simulink model "FAFA_Simulation"  (R2024b)
settings: Solver=FixedStepAuto  StartTime=0.0  StopTime=250  FixedStep=0.1  RelTol=1e-3
model workspace (MAT data in the model file):
  E = 0
  N = 0
  U = 70
  a_lat = [-2.8994 -3.7694 4.8979 0.9075 0.2017 1.1605 -2.4536 1.8506 -1.4522 0.9879 -4.2099 6.4665 ... (16 elements, 4x4)]
  a_lon = [-0.1636 0.8185 -0.1448 0.6823 -0.7164 -0.2899 -2.0395 -2.5415 0.3908 2.1971 -0.2446 -6.117 ... (16 elements, 4x4)]
  b_lat = [-2.6641  1.8404; -6.8743  1.3852; 17.3529  -0.0089; -11.8089  -3.3692]
  b_lon = [1.3105; 2.2437; -0.9608; -9.211]
  c_lat = [-0.6923 -1.1619 0.5476 -0.4273 0.0805 0.5751 0.4203 0.7792 -0.3221 1.1098 0.2079 0.2479 ... (16 elements, 4x4)]
  c_lon = [-5.1576 -0.0952 0.5331 3.6707 -28.9963 -0.3715 -3.4973 -0.1414 19.7487 -0.0997 -0.5832 -0.2256 ... (16 elements, 4x4)]
  d_lat = [0  0; 0  0; 0  0; 0  0]
  d_lon = [0; 0; 0; 0]
  psi0 = 0
  wind_E0 = 0
  wind_N0 = 0
  wind_heading = 100
  wind_noise = 0
  wind_turbulance_value0 = 1
  wind_value0 = 0
  x0_lat = [0; 0; 0; 0]
  x0_lon = [0; 0; 0; 0]
values from neighbouring files (symbols this model uses):
  velocity = zeros(num_waypoints, 3)    [training_engine.m]
  waypoints = all_waypoints    [training_engine.m]
undefined symbols (not defined in the file or in its folder): dspblkCoreblockFVToolHelper, F, gcbh, Light, MIL
libraries: simulink x8, slpidlib x5, aerolibwind2 x3, sharedtransform x2, rllib x1, uavutilslib x1
(part 3 of 3)

== matlab function FAFA_Simulation/OBSERVATION/Straight Line V4 ==
  data: waypoints_window input; velocity_window input; valid_flag input; loiter_flag input; uav_e input; global_path output size=[inf 3]; uav_n input; uav_u input; guidance_mode output; uav_phi input; uav_theta input; uav_psi input; debug_cte output; debug_curvature output
function [global_path, guidance_mode, debug_cte, debug_curvature] = guidance_function_hybrid_Straight_Line(waypoints_window, velocity_window, valid_flag, loiter_flag, uav_e, uav_n, uav_u, uav_phi, uav_theta, uav_psi)
% guidance_mode: 0=無效, 1=純B-spline, 2=SPSO+B-spline, 3=Loiter模式
%#codegen

%  Loiter 模式開關
ENABLE_LOITER = false;

persistent last_point_initialized last_point stored_global_path stored_path_length ...
           loiter_mode initialized theta_current center loiter_arc transition ...
           a1_mode_active

if isempty(last_point_initialized)
    last_point_initialized = false;
    last_point            = zeros(1,3);
    stored_global_path    = zeros(100000,3);
    stored_path_length    = 1;
    loiter_mode           = false;
    initialized = false;
    theta_current = 0;
    center = [0 0];
    loiter_arc = zeros(3,3);
    transition = false;
    a1_mode_active = false;
end

% 確保輸出在所有路徑都有明確的標量值
guidance_mode = 0;
debug_cte = 0;
debug_curvature = 0;

R = 100;
dtheta_deg = 1;
uav_position = [uav_e, uav_n, uav_u];

%% ==== Loiter 模式 ====
% 只有當 ENABLE_LOITER = true 時才會進入 Loiter 邏輯
if ENABLE_LOITER && loiter_flag && ~initialized
    if stored_path_length >= 2
        pos_prev = stored_global_path(stored_path_length-1, 1:2);
        pos_curr = stored_global_path(stored_path_length, 1:2);
        heading_vec = pos_curr - pos_prev;
        yaw = atan2(heading_vec(2), heading_vec(1));
    else
        yaw = 0;
    end

    dists = vecnorm(waypoints_window(:,1:2) - uav_position(1:2), 2, 2);
    [~, idx_nearest] = min(dists);
    P0 = waypoints_window(idx_nearest, 1:2);
    center = P0 + [cos(yaw), sin(yaw)] * R * 1.5;
    theta_current = atan2(uav_position(2) - center(2), ...
                           uav_position(1) - center(1));
    loiter_mode = true;
    initialized = true;
end

if ENABLE_LOITER && loiter_mode
    guidance_mode = 3;
    a1_mode_active = false;

    if loiter_flag
        dtheta = deg2rad(dtheta_deg);
        spacing = 1.0;
        arc_length = R * dtheta;
        num_points = max(3, ceil(arc_length / spacing));
        theta_list = theta_current - linspace(0, dtheta, num_points);
        x_list = center(1) + R * cos(theta_list);
        y_list = center(2) + R * sin(theta_list);
        z_list = repmat(uav_u, size(x_list));

        loiter_arc_raw = [x_list', y_list', z_list'];
        arc_diff = diff(loiter_arc_raw);
        arc_seg_length = sqrt(sum(arc_diff.^2, 2));
        cum_length = [0; cumsum(arc_seg_length)];
        total_length = cum_length(end);

        num_interp = max(2, ceil(total_length));
        query_dist = linspace(0, total_length, num_interp)';
        interp_x = interp1(cum_length, loiter_arc_raw(:,1), query_dist, 'linear');
        interp_y = interp1(cum_length, loiter_arc_raw(:,2), query_dist, 'linear');
        interp_z = interp1(cum_length, loiter_arc_raw(:,3), query_dist, 'linear');
        loiter_arc = [interp_x, interp_y, interp_z];
        theta_current = theta_list(end);

        if ~transition
            loiter_entry = loiter_arc(1,:);
            loiter_tangent = loiter_arc(2,1:2) - loiter_arc(1,1:2);
            loiter_tangent = loiter_tangent / (norm(loiter_tangent) + 1e-6);

            dists = vecnorm(waypoints_window(:,1:2) - uav_position(1:2), 2, 2);
            [~, idx_nearest] = min(dists);
            P0 = waypoints_window(idx_nearest, :);

            connect_tangent = loiter_entry(1:2) - P0(1:2);
            connect_tangent = connect_tangent / (norm(connect_tangent) + 1e-6);
            dist = norm(loiter_entry(1:2) - P0(1:2));

            P1 = P0(1:2) + 0.3 * dist * connect_tangent;
            P2 = loiter_entry(1:2) - 0.3 * dist * loiter_tangent;
            P3 = loiter_entry(1:2);

            t = linspace(0,1,ceil(dist));
            bezier_x = (1-t).^3 * P0(1) + 3*(1-t).^2 .* t * P1(1) + 3*(1-t).*t.^2 * P2(1) + t.^3 * P3(1);
            bezier_y = (1-t).^3 * P0(2) + 3*(1-t).^2 .* t * P1(2) + 3*(1-t).*t.^2 * P2(2) + t.^3 * P3(2);
            bezier_z = linspace(P0(3), loiter_entry(3), numel(t));
            transition_path = [bezier_x', bezier_y', bezier_z'];

            combined_path = [transition_path; loiter_arc(2:end,:)];
            global_path = combined_path;
            transition = true;
        else
            global_path = loiter_arc;
        end
        return;
    else
        % 退出 Loiter 的邏輯
        arc_exit_pt = loiter_arc(end, :);
        arc_tangent = loiter_arc(end,1:2) - loiter_arc(end-1,1:2);
        arc_tangent = arc_tangent / (norm(arc_tangent) + 1e-6);
        R_min = 55;
        dists = vecnorm(waypoints_window(:,1:2) - arc_exit_pt(1:2), 2, 2);
        [~, idx_nearest] = min(dists);
        lookahead_distance = 100;
        accum_dist = 0;
        idx_target = idx_nearest;

        while accum_dist < lookahead_distance && idx_target < size(waypoints_window,1)
            delta = norm(waypoints_window(idx_target+1,1:2) - waypoints_window(idx_target,1:2));
            accum_dist = accum_dist + delta;
            idx_target = idx_target + 1;
        end

        p_target = waypoints_window(idx_target, :);

        if idx_target < size(waypoints_window,1)
            next_vec = waypoints_window(idx_target+1,1:2) - waypoints_window(idx_target,1:2);
        else
            next_vec = waypoints_window(idx_target,1:2) - waypoints_window(idx_target-1,1:2);
        end

        target_tangent = next_vec / (norm(next_vec) + 1e-6);
        P0 = arc_exit_pt;
        P3 = p_target;
        total_dist = norm(P3(1:2) - P0(1:2));
        theta = acos(dot(arc_tangent, target_tangent));
        d_min = R_min * tan(theta/2);
        d = max(d_min, R_min);
        success = false;
        B = repmat(P0, ceil(total_dist), 1);

        while ~success && d <= total_dist
            P1 = P0 + [arc_tangent, 0] * 0.3 * d;
            P2 = P3 - [target_tangent, 0] * 0.1 * d;
            t = linspace(0,1,ceil(total_dist));
            B = (1 - t').^3 * P0 + 3*(1 - t').^2 .* t' * P1 + 3*(1 - t') .* t'.^2 * P2 + t'.^3 * P3;
            d1 = diff(B, 1, 1);
            d2 = diff(d1, 1, 1);
            cross_z = d1(1:end-1,1) .* d2(:,2) - d1(1:end-1,2) .* d2(:,1);
            curvature = abs(cross_z) ./ (vecnorm(d1(1:end-1,:),2,2).^3 + 1e-6);

            if all(1./(curvature + 1e-6) >= R_min)
                success = true;
            else
                d = d + 5;
            end
        end

        segment = B;
        stored_global_path(1:size(segment,1), :) = segment;
        stored_path_length = size(segment,1);
        loiter_mode = false;
        initialized = false;
        transition = false;
        global_path = segment;

        % 固定維度賦值
        if size(segment,1) >= 1
            last_point(1,1) = segment(end, 1);
            last_point(1,2) = segment(end, 2);
            last_point(1,3) = segment(end, 3);
        end
        return;
    end
end

%% ========== v8 混合規劃器 ==========
if valid_flag && ~loiter_mode

    N_WAYPOINTS = size(waypoints_window, 1);

    % 起點處理
    if ~last_point_initialized
        P_start_spline = [uav_e, uav_n, uav_u];
        last_point_initialized = true;
    else
        P_start_spline = last_point;
    end

    P_end = waypoints_window(end, :);

    % ====== 計算 UAV 到滑窗的真正 CTE（垂直投影距離） ======
    uav_cte = inf;
    if N_WAYPOINTS >= 2
        for i = 1:N_WAYPOINTS-1
            seg_s = waypoints_window(i, 1:2);
            seg_e = waypoints_window(i+1, 1:2);
            seg_v = seg_e - seg_s;
            seg_l = norm(seg_v);
            if seg_l < 1e-6, continue; end
            to_uav = uav_position(1:2) - seg_s;
            proj = max(0, min(1, dot(to_uav, seg_v) / (seg_l^2)));
            d = norm(uav_position(1:2) - (seg_s + proj * seg_v));
            if d < uav_cte, uav_cte = d; end
        end
    end

    % 點到點距離（用於 A-2 和 SPSO 判斷）
    dists_to_window = vecnorm(waypoints_window(:,1:2) - uav_position(1:2), 2, 2);
    [min_dist_to_window, ~] = min(dists_to_window);
    dist_start_to_window = norm(P_start_spline(1:2) - waypoints_window(1,1:2));

    % ====== 計算滑窗最大曲率 (Menger curvature) ======
    max_curvature = 0;
    if N_WAYPOINTS >= 3
        for i = 2:N_WAYPOINTS-1
            AB = waypoints_window(i,1:2) - waypoints_window(i-1,1:2);
            BC = waypoints_window(i+1,1:2) - waypoints_window(i,1:2);
            AC = waypoints_window(i+1,1:2) - waypoints_window(i-1,1:2);
            cross_z = abs(AB(1)*BC(2) - AB(2)*BC(1));
            denom = norm(AB) * norm(BC) * norm(AC);

            if denom > 1e-10
                kappa = 2 * cross_z / denom;
                if kappa > max_curvature
                    max_curvature = kappa;
                end
            end
        end
    end

    % ====== 計算滑窗平均朝向，並與 UAV 航向比較 ======
    % uav_psi 使用弧度；此處以滑窗各線段向量加總作為平均朝向
    window_avg_vec = [0, 0];
    heading_error = pi;

    if N_WAYPOINTS >= 2
        for i = 1:N_WAYPOINTS-1
            seg_vec_heading = waypoints_window(i+1, 1:2) - waypoints_window(i, 1:2);
            if norm(seg_vec_heading) > 1e-6
                window_avg_vec = window_avg_vec + seg_vec_heading;
            end
        end

        if norm(window_avg_vec) > 1e-6
            window_avg_heading = atan2(window_avg_vec(2), window_avg_vec(1));
            heading_error = atan2(sin(window_avg_heading - uav_psi), ...
                                  cos(window_avg_heading - uav_psi));
        end
    end

    CURVATURE_THRESHOLD = 0.005;   % 曲率門檻 (對應半徑 > 200m)

    % A-1 航向遲滯門檻：
    % 尚未進入 A-1 時，需小於 17 deg 才允許進入；
    % 已在 A-1 時，允許到 23 deg 才退出，避免在 20 deg 附近反覆切換。
    HEADING_ALIGNMENT_CENTER = deg2rad(20);
    HEADING_ALIGNMENT_RANGE  = deg2rad(3);
    HEADING_ENTER_THRESHOLD  = HEADING_ALIGNMENT_CENTER - HEADING_ALIGNMENT_RANGE;  % 17 deg
    HEADING_EXIT_THRESHOLD   = HEADING_ALIGNMENT_CENTER + HEADING_ALIGNMENT_RANGE;  % 23 deg

    CTE_THRESHOLD = 35;            % CTE 門檻 (m)，使用垂直投影距離
    DEVIATION_THRESHOLD = 100;

    % ====== Debug 輸出 ======
    debug_cte = uav_cte;
    debug_curvature = max_curvature;

    % ====== A-1 航向遲滯判斷 ======
    if a1_mode_active
        a1_heading_condition = abs(heading_error) <= HEADING_EXIT_THRESHOLD;
    else
        a1_heading_condition = abs(heading_error) <= HEADING_ENTER_THRESHOLD;
    end

    if max_curvature < CURVATURE_THRESHOLD && a1_heading_condition
        % ========== 模式A-1：低曲率 + 航向對齊 → 純 B-spline (從 UAV 位置出發) ==========
        guidance_mode = 1;
        a1_mode_active = true;
        N_CONTROL_POINTS = 6;
        indices = round(linspace(1, N_WAYPOINTS, N_CONTROL_POINTS));
        best_control_points = waypoints_window(indices, :);
        best_control_points(1, :) = uav_position;  % ★ 從自身位置開始

    elseif min_dist_to_window < DEVIATION_THRESHOLD && dist_start_to_window < DEVIATION_THRESHOLD
        % ========== 模式A-2：原始純 B-spline (從 last_point 出發) ==========
        guidance_mode = 1;
        a1_mode_active = false;
        N_CONTROL_POINTS = 6;
        indices = round(linspace(1, N_WAYPOINTS, N_CONTROL_POINTS));
        best_control_points = waypoints_window(indices, :);
        best_control_points(1, :) = P_start_spline;

    else
        % ========== 模式B：SPSO + B-spline ==========
        guidance_mode = 2;
        a1_mode_active = false;

        % SPSO 起點：強制為 UAV 當前位置
        P_start_SPSO = uav_position;

        % ====== 目標行駛方向（由速度滑窗估計，僅 SPSO 使用） ======
        v_tar_2d = [0, 0];
        if ~isempty(velocity_window)
            N_vel = size(velocity_window, 1);
            if N_vel >= 1
                K = min(3, N_vel);
                idx_start = N_vel - K + 1;
                v_seg = velocity_window(idx_start:N_vel, 1:2);
                v_mean = mean(v_seg, 1);
                if norm(v_mean) > 1e-3
                    v_tar_2d = v_mean;
                else
                    v_tar_2d = [0, 0];
                end
            end
        end

        % SPSO參數
        nParticles = 10;
        maxIter = 20;
        w = 0.4;
        c1 = 1.5;
        c2 = 1.5;

        N_CONTROL_POINTS = 5;
        N_OPTIMIZE = 3;

        max_segment_length = 50;
        min_segment_length = 5;
        max_climb_angle_rad = deg2rad(20);
        max_turn_angle_rad  = deg2rad(35);

        b1 = 0.6;
        b2 = 0.2;
        b3 = 0.1;
        b4 = 0.1;

        % 參考採樣
        sample_idx = round(linspace(1, N_WAYPOINTS, N_CONTROL_POINTS));
        control_waypoints = waypoints_window(sample_idx, :);

        % 初始化參考向量
        reference_vectors = control_waypoints - P_start_SPSO;
        rho_ref = vecnorm(reference_vectors, 2, 2);
        theta_ref = asin(reference_vectors(:,3) ./ (rho_ref + 1e-6));
        phi_ref = atan2(reference_vectors(:,2), reference_vectors(:,1));

        dim = N_OPTIMIZE * 3;
        particles = zeros(nParticles, dim);
        velocities = zeros(nParticles, dim);

        for i = 1:nParticles
            for j = 1:N_OPTIMIZE
                ref_idx = j + 1;
                idx = (j-1)*3 + 1;

                if i == 1
                    particles(1, idx)   = rho_ref(ref_idx);
                    particles(1, idx+1) = theta_ref(ref_idx);
                    particles(1, idx+2) = phi_ref(ref_idx);
                else
                    particles(i, idx)   = rho_ref(ref_idx) * (1 + randn() * 0.1);
                    particles(i, idx+1) = theta_ref(ref_idx) + randn() * deg2rad(2);
                    particles(i, idx+2) = phi_ref(ref_idx) + randn() * deg2rad(5);
                end

                particles(i, idx) = max(min_segment_length, min(particles(i, idx), max_segment_length));
                particles(i, idx+1) = max(-max_climb_angle_rad, min(particles(i, idx+1), max_climb_angle_rad));

                if j == 1
                    base_heading = uav_psi;
                else
                    prev_phi_idx = (j-2)*3 + 3;
                    base_heading = particles(i, prev_phi_idx);
                end

                dphi = particles(i, idx+2) - base_heading;
                dphi = mod(dphi + pi, 2*pi) - pi;
                if dphi > max_turn_angle_rad
                    dphi = max_turn_angle_rad;
                elseif dphi < -max_turn_angle_rad
                    dphi = -max_turn_angle_rad;
                end
                particles(i, idx+2) = mod(base_heading + dphi + pi, 2*pi) - pi;
            end
            velocities(i, :) = randn(1, dim) * 0.01;
        end

        % SPSO迭代
        fitness = zeros(nParticles, 1);
        for i = 1:nParticles
            fitness(i) = evaluateFitness_CostStruct(particles(i,:), P_start_SPSO, P_end, ...
                          control_waypoints, N_CONTROL_POINTS, b1, b2, b3, b4, ...
                          uav_psi, v_tar_2d);
        end

        [~, best_idx] = min(fitness);
        personal_best = particles;
        personal_best_fitness = fitness;
        global_best = particles(best_idx, :);
        global_best_fitness = fitness(best_idx);

        for iter = 1:maxIter
            for i = 1:nParticles
                r1 = rand(1, dim);
                r2 = rand(1, dim);
                velocities(i,:) = w * velocities(i,:) + ...
                                  c1 * r1 .* (personal_best(i,:) - particles(i,:)) + ...
                                  c2 * r2 .* (global_best - particles(i,:));
                particles(i,:) = particles(i,:) + velocities(i,:);

                for j = 1:N_OPTIMIZE
                    idx = (j-1)*3 + 1;
                    particles(i, idx) = max(min_segment_length, min(particles(i, idx), max_segment_length));
                    particles(i, idx+1) = max(-max_climb_angle_rad, min(particles(i, idx+1), max_climb_angle_rad));

                    phi_idx = idx + 2;
                    if j == 1
                        base_heading = uav_psi;
                    else
                        prev_phi_idx = (j-2)*3 + 3;
                        base_heading = particles(i, prev_phi_idx);
                    end

                    dphi = particles(i, phi_idx) - base_heading;
                    dphi = mod(dphi + pi, 2*pi) - pi;
                    if dphi > max_turn_angle_rad
                        dphi = max_turn_angle_rad;
                    elseif dphi < -max_turn_angle_rad
                        dphi = -max_turn_angle_rad;
                    end
                    particles(i, phi_idx) = mod(base_heading + dphi + pi, 2*pi) - pi;
                end

                fitness(i) = evaluateFitness_CostStruct(particles(i,:), P_start_SPSO, P_end, ...
                              control_waypoints, N_CONTROL_POINTS, b1, b2, b3, b4, ...
                              uav_psi, v_tar_2d);

                if fitness(i) < personal_best_fitness(i)
                    personal_best(i,:) = particles(i,:);
                    personal_best_fitness(i) = fitness(i);
                end
            end

            [current_best_fitness, best_idx] = min(fitness);
            if current_best_fitness < global_best_fitness
                global_best = particles(best_idx, :);
                global_best_fitness = current_best_fitness;
            end
        end

        % 構建最終控制點
        best_control_points = zeros(N_CONTROL_POINTS, 3);
        best_control_points(1, :) = P_start_SPSO;
        best_control_points(end, :) = P_end;

        for j = 1:N_OPTIMIZE
            idx = (j-1)*3 + 1;
            rho   = global_best(idx);
            theta = global_best(idx+1);
            phi   = global_best(idx+2);
            dx = rho * cos(theta) * cos(phi);
            dy = rho * cos(theta) * sin(phi);
            dz = rho * sin(theta);
            best_control_points(j+1, :) = best_control_points(j, :) + [dx, dy, dz];
        end
    end

    % 生成 B-spline
    N_samples = 100;
    path_smooth = generate_Bspline(best_control_points, N_samples);

    % Resample
    segment_diff = diff(path_smooth);
    segment_length = sqrt(sum(segment_diff.^2, 2));
    cumulative_length = [0; cumsum(segment_length)];
    total_length = cumulative_length(end);

    if total_length < 1e-3
        if stored_path_length > 1
             global_path = stored_global_path(1:stored_path_length,:);
        else
             global_path = path_smooth;
        end
        return;
    end

    desired_spacing = 1;
    num_new_points = max(2, floor(total_length / desired_spacing));
    query_distances = linspace(0, total_length, num_new_points)';

    interp_x = interp1(cumulative_length, path_smooth(:,1), query_distances, 'linear');
    interp_y = interp1(cumulative_length, path_smooth(:,2), query_distances, 'linear');
    interp_z = interp1(cumulative_length, path_smooth(:,3), query_distances, 'linear');

    new_path = [interp_x, interp_y, interp_z];
    stored_global_path(:,:) = 0;

    if isempty(new_path)
        stored_global_path(1:size(best_control_points,1),:) = best_control_points;
        stored_path_length = size(best_control_points,1);
        last_point(1,1) = best_control_points(end, 1);
        last_point(1,2) = best_control_points(end, 2);
        last_point(1,3) = best_control_points(end, 3);
    else
        stored_global_path(1:size(new_path,1),:) = new_path;
        stored_path_length = size(new_path,1);
        last_point(1,1) = new_path(end, 1);
        last_point(1,2) = new_path(end, 2);
        last_point(1,3) = new_path(end, 3);
    end
end

global_path = stored_global_path(1:stored_path_length,:);
end

%% ========== B-spline生成器 ==========
function path_smooth = generate_Bspline(control_points, num_samples)
    N = size(control_points, 1);
    if N < 2
        path_smooth = control_points;
        return;
    end
    segment_lengths = sqrt(sum(diff(control_points).^2, 2));
    t_control = [0; cumsum(segment_lengths)];
    valid_idx = [true; segment_lengths > 1e-6];
    if sum(valid_idx) < 2
        path_smooth = repmat(control_points(1,:), num_samples, 1);
        return;
    end
    t_control_valid = t_control(valid_idx);
    control_points_valid = control_points(valid_idx, :);
    if isempty(t_control_valid) || t_control_valid(end) < 1e-6
        path_smooth = repmat(control_points(1,:), num_samples, 1);
        return;
    end
    t_control_valid = t_control_valid / t_control_valid(end);
    t_query = linspace(0, 1, num_samples)';
    x_smooth = spline(t_control_valid, control_points_valid(:,1), t_query);
    y_smooth = spline(t_control_valid, control_points_valid(:,2), t_query);
    z_smooth = spline(t_control_valid, control_points_valid(:,3), t_query);
    path_smooth = [x_smooth, y_smooth, z_smooth];
end

%% ========== Cost Function（含終端入射角約束） ==========
function cost = evaluateFitness_CostStruct(particle, P_start, P_end, control_waypoints, N_control, ...
                                           b1, b2, b3, b4, ...
                                           uav_psi, v_tar_2d)
    % 1. 重建路徑
    path = zeros(N_control, 3);
    path(1, :) = P_start;
    path(end, :) = P_end;

    N_optimize = (N_control - 2);
    for j = 1:N_optimize
        idx = (j-1)*3 + 1;
        rho   = particle(idx);
        theta = particle(idx+1);
        phi   = particle(idx+2);
        dx = rho * cos(theta) * cos(phi);
        dy = rho * cos(theta) * sin(phi);
        dz = rho * sin(theta);
        path(j+1, :) = path(j, :) + [dx, dy, dz];
    end

    % ========== F1: 路徑長度成本 ==========
    path_diff = diff(path);
    segment_lengths = sqrt(sum(path_diff.^2, 2));
    total_length = sum(segment_lengths);
    straight_dist = norm(P_end - P_start);

    if straight_dist > 1e-6
        F1 = total_length / straight_dist;
        F1 = min(F1, 3.0);
    else
        F1 = 1.0;
    end

    % ========== F2: 路徑跟隨成本 ==========
    F2_raw = 0;
    for i = 1:size(path,1)
        dists = vecnorm(control_waypoints - path(i,:), 2, 2);
        [min_dist, ~] = min(dists);
        F2_raw = F2_raw + min_dist^2;
    end
    F2 = F2_raw / (size(path,1) * 100);
    F2 = min(F2, 10.0);

    % ========== F3: 平滑度成本 ==========
    F3_raw = 0;
    max_turn_angle = deg2rad(35);

    % (A) 第一段 vs UAV 航向
    vec_first = path(2,1:2) - path(1,1:2);
    if norm(vec_first) > 1e-6
        current_psi_vec = [cos(uav_psi), sin(uav_psi)];
        dot_val = dot(vec_first/norm(vec_first), current_psi_vec);
        angle_diff_start = acos(max(-1, min(1, dot_val)));
        if angle_diff_start > max_turn_angle
            cost = 1e9;
            return;
        end
        F3_raw = F3_raw + angle_diff_start;
    end

    % (B) 後續段之間的夾角
    for i = 1:size(path,1)-2
        v1 = path(i+1,1:2) - path(i,1:2);
        v2 = path(i+2,1:2) - path(i+1,1:2);
        if norm(v1) > 1e-6 && norm(v2) > 1e-6
            dot_prod = dot(v1, v2);
            cross_prod = v1(1)*v2(2) - v1(2)*v2(1);
            phi_turn = atan2(cross_prod, dot_prod);
            if abs(phi_turn) > max_turn_angle
                cost = 1e9;
                return;
            end
            F3_raw = F3_raw + abs(phi_turn);
        end
    end
    F3 = F3_raw;

    % ========== F4: 終點誤差成本 ==========
    endpoint_error = norm(path(end,:) - P_end);
    if endpoint_error > 20
        cost = 1e9 + endpoint_error * 1000;
        return;
    end
    F4 = endpoint_error / 10.0;

    % ========== F5: 終端入射角約束 ==========
    if ~(v_tar_2d(1) == 0 && v_tar_2d(2) == 0)
        if size(path,1) < 2
            cost = 1e9;
            return;
        end

        v_last = path(end,1:2) - path(end-1,1:2);
        if norm(v_last) < 1e-6
            cost = 1e9;
            return;
        end
        v_last = v_last / norm(v_last);

        v_tar = v_tar_2d;
        if norm(v_tar) < 1e-6
            % 不啟用此約束
        else
            v_tar = v_tar / norm(v_tar);
            dot_val   = dot(v_last, v_tar);
            dot_val   = max(-1, min(1, dot_val));
            cross_val = v_last(1)*v_tar(2) - v_last(2)*v_tar(1);
            delta_psi_entry = atan2(cross_val, dot_val);

            max_entry = deg2rad(45);
            if abs(delta_psi_entry) > max_entry
                cost = 1e9;
                return;
            end
        end
    end

    % ========== 總成本 ==========
    cost = b1*F1 + b2*F2 + b3*F3 + b4*F4;

    if isnan(cost) || isinf(cost)
        cost = 1e10;
    end
end

== matlab function FAFA_Simulation/OBSERVATION/MATLAB Function20 ==
  data: bool input; y output
function y = fcn(bool)
if bool == 0
    y = 0;
else
    y = -0.1;
end

== matlab function FAFA_Simulation/OBSERVATION/MATLAB Function21 ==
  data: d input; y output
% function y = fcn(d, dis)
%     if isempty(dis)
%         y = 0;
%     end
%     if dis <= 150 && dis >= 30
%         a = 0.5;
%     else
%         a = 0;
%     end
%     if d <= 10
%         b = 0.5;
%     else
%         b = 0;
%     end
%     y = a+b;
% 
% end
    
function y = fcn(d)
    if d <= 10
        b = 0.5;
    else
        b = 0;
    end
    y = b;

end

== matlab function FAFA_Simulation/OBSERVATION/MATLAB Function22 ==
  data: d input; dis input; y output
function y = fcn(d, dis)
    if isempty(dis)
        y = 0;
    end
    if dis <= 150 && dis >= 30
        a = 0.5;
    else
        a = 0;
    end
    if d <= 10
        b = 0.5;
    else
        b = 0;
    end
    y = a+b;

end



% function y = fcn(d, dis)
%     % 漸進式獎勵：d和dis都使用平滑函數
%     if isempty(dis)
%         y = 0;
%         return;
%     end
% 
%     % ========== 條件A：距離獎勵（高斯函數） ==========
%     % 最佳距離: 60m，允許範圍: 20~150m
%     d_optimal = 60;
%     d_tolerance = 50;  % 標準差
% 
%     % 使用高斯函數：距離d_optimal越近獎勵越高
%     a = 0.5 * exp(-((dis - d_optimal)^2) / (2 * d_tolerance^2));
% 
%     % 硬約束：超出20~200m範圍直接歸零
%     if dis < 20 || dis > 200
%         a = 0;
%     end
% 
%     % ========== 條件B：橫向誤差獎勵（反比函數） ==========
%     % d越小獎勵越高，使用平滑的反比函數
%     d_threshold = 30;  % 20m以內都有獎勵
% 
%     if d <= d_threshold
%         % 使用平滑的反比函數
%         b = 0.5 * (1 - (d / d_threshold)^2);
%     else
%         b = 0;
%     end
% 
%     % ========== 總獎勵 ==========
%     y = a + b;
% 
%     % 限制範圍在[0, 1]
%     y = max(0, min(1, y));
% end

== matlab function FAFA_Simulation/OBSERVATION/MATLAB Function2 ==
  data: x input; y output; finite input
function y = Normalization(x,finite)
y = (x-(-finite))/(finite-(-finite))*2-1;

== matlab function FAFA_Simulation/OBSERVATION/MATLAB Function3 ==
  data: position_in input; waypoints_window output size=[inf 3]; velocity_in input; window_length input; velocity_window output size=[inf 3]; valid_flag output; loiter_flag output; uav_e input; uav_n input; distance_to_target output
function [waypoints_window, velocity_window, valid_flag, loiter_flag, distance_to_target] = WindowManager(position_in, velocity_in, window_length, uav_e, uav_n)
%#codegen
% Spatial route following: monotonic progress and contiguous forward chunks.
persistent progress last_emitted
if isempty(progress), progress=1; last_emitted=0; end
waypoints_window=zeros(window_length,3); velocity_window=zeros(window_length,3);
valid_flag=false; loiter_flag=false; distance_to_target=0;
n=size(position_in,1);
if n<window_length, return; end
best=progress; best_d=Inf;
for k=progress:min(n,progress+window_length)
 d=(position_in(k,1)-uav_e)^2+(position_in(k,2)-uav_n)^2;
 if d<best_d, best_d=d; best=k; end
end
progress=best; first=max(1,last_emitted);
if last_emitted==0
 valid_flag=true;
elseif progress>=last_emitted+window_length-1-40 && last_emitted+2*(window_length-1)<=n
 first=last_emitted+window_length-1; valid_flag=true;
end
waypoints_window=position_in(first:first+window_length-1,:);
velocity_window=velocity_in(first:first+window_length-1,:);
distance_to_target=sqrt(best_d);
if valid_flag, last_emitted=first; end
end

== matlab function FAFA_Simulation/OBSERVATION/MATLAB Function5 ==
  settings: updateMethod=DISCRETE
  data: P_E input; P_E_norm output; P_N input; P_U input; alpha input; P_N_norm output
function [P_E_norm, P_N_norm] = dynamicNormalization(P_E, P_N, P_U, alpha)
    % 動態標準化函數 (Exponential Moving Normalization)
    % 輸入:
    %   P_E, P_N, P_U: 當前無人機位置
    %   alpha: 更新速率 (0.001 - 0.01)
    % 輸出:
    %   P_E_norm, P_N_norm, P_U_norm: 標準化後的數據

    % 記憶變量 (持續性變量)
    persistent mu_x sigma_x mu_y sigma_y mu_z sigma_z;

    % 初始化均值和標準差
    if isempty(mu_x)
        mu_x = 0; sigma_x = 10;
        mu_y = 0; sigma_y = 10;
        mu_z = 0; sigma_z = 10;
    end

    % 更新均值 (Exponential Moving Average)
    mu_x = (1 - alpha) * mu_x + alpha * P_E;
    mu_y = (1 - alpha) * mu_y + alpha * P_N;
    mu_z = (1 - alpha) * mu_z + alpha * P_U;

    % 更新標準差 (Exponential Moving Variance)
    sigma_x = sqrt((1 - alpha) * sigma_x^2 + alpha * (P_E - mu_x)^2 + 1e-6);
    sigma_y = sqrt((1 - alpha) * sigma_y^2 + alpha * (P_N - mu_y)^2 + 1e-6);
    sigma_z = sqrt((1 - alpha) * sigma_z^2 + alpha * (P_U - mu_z)^2 + 1e-6);

    % 設定最小標準差，防止標準差過小
    sigma_min = 1e-2;  % 避免標準化後數值過大
    sigma_x = max(sigma_x, sigma_min);
    sigma_y = max(sigma_y, sigma_min);
    sigma_z = max(sigma_z, sigma_min);

    % 標準化輸出
    P_E_norm = (P_E - mu_x) / sigma_x;
    P_N_norm = (P_N - mu_y) / sigma_y;
    P_U_norm = (P_U - mu_z) / sigma_z;

    % 限制範圍 (-3, 3)
    P_E_norm = max(min(P_E_norm, 3), -3);
    P_N_norm = max(min(P_N_norm, 3), -3);
    % P_U_norm = max(min(P_U_norm, 3), -3);
end

== matlab function FAFA_Simulation/OBSERVATION/MATLAB Function1 ==
  data: x input; y output; finite input
function y = Normalization(x,finite)
y = (x-(-finite))/(finite-(-finite))*2-1;

== matlab function FAFA_Simulation/OBSERVATION/MATLAB Function4 ==
  data: x input; y output; finite input
function y = Normalization(x,finite)
y = (x-(-finite))/(finite-(-finite))*2-1;
